simulink model "example_1"  (R2022b)
settings: Solver=VariableStepAuto  StartTime=0.0  StopTime=5  RelTol=1e-3
InitFcn:
  | %% Motor parameter
  | R = 0.6; % (Ohms) Resistance
  | L = 1.5e-03; % (H) Inductance
  | % Controller
  | k = 1/R;
  | wBW = 2*pi*1000;
  | Ti = L/R;
  | Kp = wBW*Ti/k;
  | Ki = Kp / Ti;
  | fs = 1e+5;
  | Ts = 1/fs;
  | wn = 2*pi*2000*10;
  | %wn = 5*wBW;
settings Model: Creator=hoang  LastModifiedBy=hoang

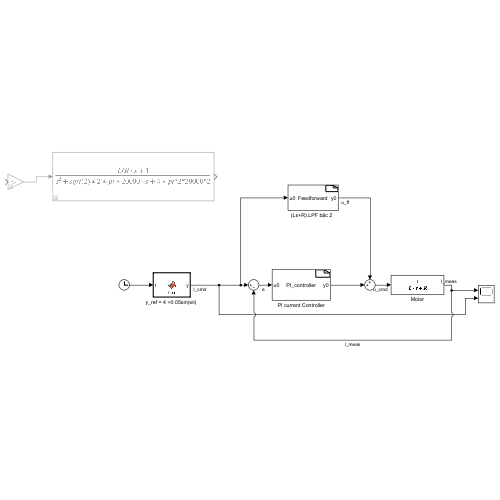
[thumbnail: Simulink's stored preview of the top-level diagram]
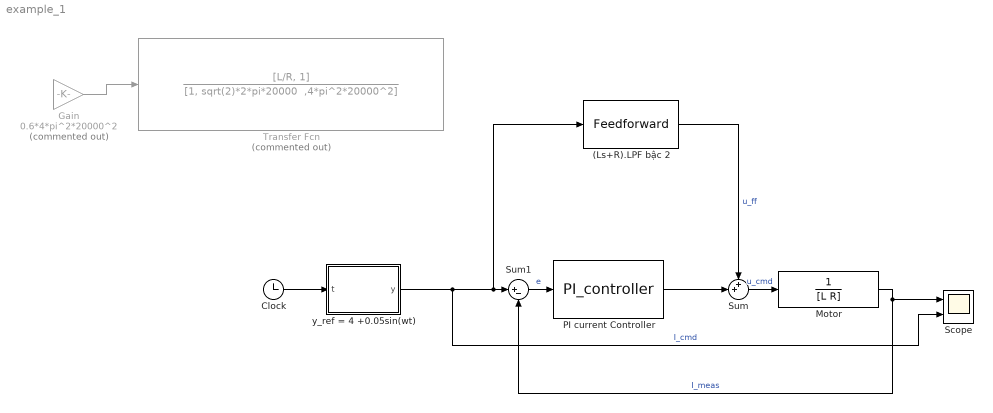
== system example_1 ==
  "(Ls+R).LPF bậc 2  " : S-Function  FunctionName=Feedforward  Parameters=L,Ts,R,wn  SFunctionModules=Feedforward_wrapper.c  SFunctionDeploymentMode=off  EnableBusSupport=off  mask(S-Function Builder){}
      mask help: Simulink:masks:SFunctionBuilder_MD
      mask init:
      | val = [[.9  0.75 0.75 1 1 .9 .9 1]',[1 1 0.75 0.75 .9 .9 1 .9]'];try , sys = get_param(gcb,'SfunBuilderFcnName');if isempty(sys), sys = get_param(gcb,'FunctionName'); end,catch, sys = get_param(gcb,'FunctionName'); end
      settings: CopyFcn=set_param(gcbh,'LinkStatus','none')  OpenFcn=sfunctionwizard(gcbh)
      mask Display:
      | plot(val(:,1),val(:,2))
      | disp(sys)
      | port_label('input',1,'u0')
      | port_label('output',1,'y0')
  Clock : Clock
  Gain : Gain  Commented=on  Gain=0.6*4*pi^2*20000^2
  Motor : TransferFcn  Denominator=[L R]
  PI current Controller : S-Function  FunctionName=PI_controller  Parameters=Ki,Kp,Ts  SFunctionModules=PI_controller_wrapper.c  SFunctionDeploymentMode=off  EnableBusSupport=off  mask(S-Function Builder){}
      mask help: Simulink:masks:SFunctionBuilder_MD
      mask init: same as example_1/(Ls+R).LPF bậc 2  
      settings: CopyFcn=set_param(gcbh,'LinkStatus','none')  OpenFcn=sfunctionwizard(gcbh)
      mask Display:
      | plot(val(:,1),val(:,2))
      | disp(sys)
      | port_label('input',1,'u0')
      | port_label('output',1,'y0')
  Scope : Scope  NumInputPorts=2
  Sum : Sum  Inputs=++|
  Sum1 : Sum  Inputs=|+-
  Transfer Fcn : TransferFcn  Commented=on  Numerator=[L/R, 1]  Denominator="[1, sqrt(2)*2*pi*20000  ,4*pi^2*20000^2]"
  "y_ref = 4 +0.05sin(wt) " : MATLAB Function  TreatAsAtomicUnit=on
  wires:
  Sum/1 -> Motor/1  "u_cmd"
  Motor/1 -> Sum1/2, Scope/1  "I_meas"
  "y_ref = 4 +0.05sin(wt) "/1(y) -> Scope/2, "(Ls+R).LPF bậc 2  "/1, Sum1/1  "I_cmd"
  Sum1/1 -> PI current Controller/1  "e"
  PI current Controller/1 -> Sum/2
  Clock/1 -> "y_ref = 4 +0.05sin(wt) "/1(t)
  Gain/1 -> Transfer Fcn/1
  "(Ls+R).LPF bậc 2  "/1 -> Sum/1  "u_ff"

== matlab function example_1/y_ref = 4 +0.05sin(wt)  ==
  data: t input; y output
function y = fcn(t)
    if (t < 1)
        y = 0;
    else 
    y = 4 + 0.5 * sin(2*pi*2000*t);
    end
end
